simulink model "r2_b8a4x1kf"  (R2012b)
settings: Solver=VariableStepDiscrete  SolverMode=SingleTasking  StartTime=0.0  StopTime=1  RelTol=1e-3
undefined symbols (not defined in the file): fft_stages, n_bits_ants, n_bits_xengs
libraries: xbsIndex_r4 x22142, casper_library_misc x166, xbsReplacements_r4 x24, casper_library_delays x8, xps_library x5, casper_library_communications x4
(part 130 of 178)

== system r2_b8a4x1kf/sys3/xeng/baseline_tap3/dual_pol_cmac/cmac2 ==
  a+bi : Inport
  c+di : Inport  Port=2
  acc_in : Inport  Port=3
  sync : Inport  Port=4
  valid_in : Inport  Port=5
  Constant1 : xbsIndex_r4/Constant  const=0  gui_display_data_type=Fixed-point  arith_type=Unsigned  n_bits=bit_growth  bin_pt=0  preci_type=Single  exp_width=8  frac_width=24  explicit_period=on  period=1  equ=P=C  opselect=C  inp2=PCIN>>17  opr=+  inp1=P  carry=CIN  dbl_ovrd=off  block_type=constant
      settings: block_version=9.2.01
  Constant2 : xbsIndex_r4/Constant  const=0  gui_display_data_type=Fixed-point  arith_type=Unsigned  n_bits=1  bin_pt=0  preci_type=Single  exp_width=8  frac_width=24  explicit_period=off  period=1  equ=P=C  opselect=C  inp2=PCIN>>17  opr=+  inp1=P  carry=CIN  dbl_ovrd=off  block_type=constant
      settings: block_version=9.2.01
  Counter : xbsIndex_r4/Counter  cnt_type=Count Limited  cnt_to=acc_len - 1  operation=Up  start_count=0  cnt_by_val=1  arith_type=Unsigned  n_bits=bit_growth  bin_pt=0  load_pin=off  rst=on  en=off  explicit_period=off  period=1  dbl_ovrd=off  use_behavioral_HDL=off  implementation=Fabric  use_rpm=on  block_type=counter
      settings: xl_area=[0, 0, 0, 0, 0, 0, 0]  block_version=9.2.01
  Delay : xbsIndex_r4/Delay  rst=off  infoeditControl=Selection of Reset will increase slice count due to use of real FFs and instead of SRLs  en=off  latency=add_latency + mult_latency - 1  dbl_ovrd=off  reg_retiming=on  block_type=delay
      settings: xl_area=[0, 0, 0, 0, 0, 0, 0]  block_version=9.2.01
  Relational : xbsIndex_r4/Relational  mode=a=b  en=off  latency=1  dbl_ovrd=off  block_type=relational
      settings: xl_area=[0, 0, 0, 0, 0, 0, 0]  block_version=9.2.01
  Terminator : Terminator
  acc : Subsystem
  acc1 : Subsystem
  c_to_ri1 : Subsystem
  c_to_ri2 : Subsystem
  cmult* : Subsystem  AncestorBlock=casper_library_multipliers/cmult  mask(cmult){n_bits_a=8, bin_pt_a=7, n_bits_b=8, bin_pt_b=7, n_bits_ab=25, bin_pt_ab=14, quantization=Truncate, overflow=Wrap, in_latency=0, mult_latency=4, add_latency=3, conv_latency=0, conjugated=on, async=off, pipelined_enable=on, multiplier_implementation=embedded multiplier core}
      mask prompts: n_bits_a "Number of Bits 'a'"; bin_pt_a "Binary Point 'a'"; n_bits_b "Number of Bits 'b'"; bin_pt_b "Binary Point 'b'"; n_bits_ab "Number of Bits 'ab'"; bin_pt_ab "Binary Point 'ab'"; in_latency "Input latency"; mult_latency "Multiplier Latency"; add_latency "Adder Latency"; conv_latency "Convert latency"; conjugated "Conjugate"; async "asynchronous operation"; pipelined_enable "enable pipeline"; multiplier_implementation "Multiplier implementation"
      mask help:
      | Multiplies two complex numbers using 4 multipliers and 2 adders.
      | Conjugation is optional.
      mask init: same as r2_b8a4x1kf/sys0/xeng/auto_tap/dual_pol_cmac/cmac1/cmult*
      settings: AttributesFormatString=|
      | 8_7 * 8_7 ==> 25_14
      | Truncate, Wrap
      | Latency=0
      mask TypeOptions quantization: Truncate | Round  (unbiased: +/- Inf) | Round  (unbiased: Even Values)
      mask TypeOptions overflow: Wrap | Saturate | Flag as error
      mask TypeOptions multiplier_implementation: behavioral HDL | standard core | embedded multiplier core
  ri_to_c : Subsystem
  acc_out : Outport
  valid_out : Outport  Port=2
  wires:
  cmult*/1(ab) -> c_to_ri1/1(In1)
  valid_in/1 -> acc1/4(valid_in)
  acc1/2(valid_out) -> valid_out/1
  acc/2(valid_out) -> Terminator/1
  Constant2/1 -> acc/4(valid_in)
  Delay/1 -> Counter/1
  sync/1 -> Delay/1
  Constant1/1 -> Relational/2
  Counter/1 -> Relational/1
  Relational/1 -> acc1/1(rst), acc/1(rst)
  c_to_ri2/2(Out2) -> acc1/3(acc_in)
  ri_to_c/1(Out1) -> acc_out/1
  acc1/1(acc_out) -> ri_to_c/2(In2)
  acc_in/1 -> c_to_ri2/1(In1)
  c+di/1 -> cmult*/2(b)
  a+bi/1 -> cmult*/1(a)
  c_to_ri1/1(Out1) -> acc/2(din)  "auto_real"
  c_to_ri1/2(Out2) -> acc1/2(din)
  acc/1(acc_out) -> ri_to_c/1(In1)
  c_to_ri2/1(Out1) -> acc/3(acc_in)

== system r2_b8a4x1kf/sys3/xeng/baseline_tap3/dual_pol_cmac/cmac3 ==
  a+bi : Inport
  c+di : Inport  Port=2
  acc_in : Inport  Port=3
  sync : Inport  Port=4
  valid_in : Inport  Port=5
  Constant1 : xbsIndex_r4/Constant  const=0  gui_display_data_type=Fixed-point  arith_type=Unsigned  n_bits=bit_growth  bin_pt=0  preci_type=Single  exp_width=8  frac_width=24  explicit_period=on  period=1  equ=P=C  opselect=C  inp2=PCIN>>17  opr=+  inp1=P  carry=CIN  dbl_ovrd=off  block_type=constant
      settings: block_version=9.2.01
  Constant2 : xbsIndex_r4/Constant  const=0  gui_display_data_type=Fixed-point  arith_type=Unsigned  n_bits=1  bin_pt=0  preci_type=Single  exp_width=8  frac_width=24  explicit_period=off  period=1  equ=P=C  opselect=C  inp2=PCIN>>17  opr=+  inp1=P  carry=CIN  dbl_ovrd=off  block_type=constant
      settings: block_version=9.2.01
  Counter : xbsIndex_r4/Counter  cnt_type=Count Limited  cnt_to=acc_len - 1  operation=Up  start_count=0  cnt_by_val=1  arith_type=Unsigned  n_bits=bit_growth  bin_pt=0  load_pin=off  rst=on  en=off  explicit_period=off  period=1  dbl_ovrd=off  use_behavioral_HDL=off  implementation=Fabric  use_rpm=on  block_type=counter
      settings: xl_area=[0, 0, 0, 0, 0, 0, 0]  block_version=9.2.01
  Delay : xbsIndex_r4/Delay  rst=off  infoeditControl=Selection of Reset will increase slice count due to use of real FFs and instead of SRLs  en=off  latency=add_latency + mult_latency - 1  dbl_ovrd=off  reg_retiming=on  block_type=delay
      settings: xl_area=[0, 0, 0, 0, 0, 0, 0]  block_version=9.2.01
  Relational : xbsIndex_r4/Relational  mode=a=b  en=off  latency=1  dbl_ovrd=off  block_type=relational
      settings: xl_area=[0, 0, 0, 0, 0, 0, 0]  block_version=9.2.01
  Terminator : Terminator
  acc : Subsystem
  acc1 : Subsystem
  c_to_ri1 : Subsystem
  c_to_ri2 : Subsystem
  cmult* : Subsystem  AncestorBlock=casper_library_multipliers/cmult  mask(cmult){n_bits_a=8, bin_pt_a=7, n_bits_b=8, bin_pt_b=7, n_bits_ab=25, bin_pt_ab=14, quantization=Truncate, overflow=Wrap, in_latency=0, mult_latency=4, add_latency=3, conv_latency=0, conjugated=on, async=off, pipelined_enable=on, multiplier_implementation=embedded multiplier core}
      mask prompts: n_bits_a "Number of Bits 'a'"; bin_pt_a "Binary Point 'a'"; n_bits_b "Number of Bits 'b'"; bin_pt_b "Binary Point 'b'"; n_bits_ab "Number of Bits 'ab'"; bin_pt_ab "Binary Point 'ab'"; in_latency "Input latency"; mult_latency "Multiplier Latency"; add_latency "Adder Latency"; conv_latency "Convert latency"; conjugated "Conjugate"; async "asynchronous operation"; pipelined_enable "enable pipeline"; multiplier_implementation "Multiplier implementation"
      mask help:
      | Multiplies two complex numbers using 4 multipliers and 2 adders.
      | Conjugation is optional.
      mask init: same as r2_b8a4x1kf/sys0/xeng/auto_tap/dual_pol_cmac/cmac1/cmult*
      settings: AttributesFormatString=|
      | 8_7 * 8_7 ==> 25_14
      | Truncate, Wrap
      | Latency=0
      mask TypeOptions quantization: Truncate | Round  (unbiased: +/- Inf) | Round  (unbiased: Even Values)
      mask TypeOptions overflow: Wrap | Saturate | Flag as error
      mask TypeOptions multiplier_implementation: behavioral HDL | standard core | embedded multiplier core
  ri_to_c : Subsystem
  acc_out : Outport
  valid_out : Outport  Port=2
  wires:
  cmult*/1(ab) -> c_to_ri1/1(In1)
  valid_in/1 -> acc1/4(valid_in)
  acc1/2(valid_out) -> valid_out/1
  acc/2(valid_out) -> Terminator/1
  Constant2/1 -> acc/4(valid_in)
  Delay/1 -> Counter/1
  sync/1 -> Delay/1
  Constant1/1 -> Relational/2
  Counter/1 -> Relational/1
  Relational/1 -> acc1/1(rst), acc/1(rst)
  c_to_ri2/2(Out2) -> acc1/3(acc_in)
  ri_to_c/1(Out1) -> acc_out/1
  acc1/1(acc_out) -> ri_to_c/2(In2)
  acc_in/1 -> c_to_ri2/1(In1)
  c+di/1 -> cmult*/2(b)
  a+bi/1 -> cmult*/1(a)
  c_to_ri1/1(Out1) -> acc/2(din)  "auto_real"
  c_to_ri1/2(Out2) -> acc1/2(din)
  acc/1(acc_out) -> ri_to_c/1(In1)
  c_to_ri2/1(Out1) -> acc/3(acc_in)

== system r2_b8a4x1kf/sys3/xeng/baseline_tap3/dual_pol_cmac/cmac4 ==
  a+bi : Inport
  c+di : Inport  Port=2
  acc_in : Inport  Port=3
  sync : Inport  Port=4
  valid_in : Inport  Port=5
  Constant1 : xbsIndex_r4/Constant  const=0  gui_display_data_type=Fixed-point  arith_type=Unsigned  n_bits=bit_growth  bin_pt=0  preci_type=Single  exp_width=8  frac_width=24  explicit_period=on  period=1  equ=P=C  opselect=C  inp2=PCIN>>17  opr=+  inp1=P  carry=CIN  dbl_ovrd=off  block_type=constant
      settings: block_version=9.2.01
  Constant2 : xbsIndex_r4/Constant  const=0  gui_display_data_type=Fixed-point  arith_type=Unsigned  n_bits=1  bin_pt=0  preci_type=Single  exp_width=8  frac_width=24  explicit_period=off  period=1  equ=P=C  opselect=C  inp2=PCIN>>17  opr=+  inp1=P  carry=CIN  dbl_ovrd=off  block_type=constant
      settings: block_version=9.2.01
  Counter : xbsIndex_r4/Counter  cnt_type=Count Limited  cnt_to=acc_len - 1  operation=Up  start_count=0  cnt_by_val=1  arith_type=Unsigned  n_bits=bit_growth  bin_pt=0  load_pin=off  rst=on  en=off  explicit_period=off  period=1  dbl_ovrd=off  use_behavioral_HDL=off  implementation=Fabric  use_rpm=on  block_type=counter
      settings: xl_area=[0, 0, 0, 0, 0, 0, 0]  block_version=9.2.01
  Delay : xbsIndex_r4/Delay  rst=off  infoeditControl=Selection of Reset will increase slice count due to use of real FFs and instead of SRLs  en=off  latency=add_latency + mult_latency - 1  dbl_ovrd=off  reg_retiming=on  block_type=delay
      settings: xl_area=[0, 0, 0, 0, 0, 0, 0]  block_version=9.2.01
  Relational : xbsIndex_r4/Relational  mode=a=b  en=off  latency=1  dbl_ovrd=off  block_type=relational
      settings: xl_area=[0, 0, 0, 0, 0, 0, 0]  block_version=9.2.01
  Terminator : Terminator
  acc : Subsystem
  acc1 : Subsystem
  c_to_ri1 : Subsystem
  c_to_ri2 : Subsystem
  cmult* : Subsystem  AncestorBlock=casper_library_multipliers/cmult  mask(cmult){n_bits_a=8, bin_pt_a=7, n_bits_b=8, bin_pt_b=7, n_bits_ab=25, bin_pt_ab=14, quantization=Truncate, overflow=Wrap, in_latency=0, mult_latency=4, add_latency=3, conv_latency=0, conjugated=on, async=off, pipelined_enable=on, multiplier_implementation=embedded multiplier core}
      mask prompts: n_bits_a "Number of Bits 'a'"; bin_pt_a "Binary Point 'a'"; n_bits_b "Number of Bits 'b'"; bin_pt_b "Binary Point 'b'"; n_bits_ab "Number of Bits 'ab'"; bin_pt_ab "Binary Point 'ab'"; in_latency "Input latency"; mult_latency "Multiplier Latency"; add_latency "Adder Latency"; conv_latency "Convert latency"; conjugated "Conjugate"; async "asynchronous operation"; pipelined_enable "enable pipeline"; multiplier_implementation "Multiplier implementation"
      mask help:
      | Multiplies two complex numbers using 4 multipliers and 2 adders.
      | Conjugation is optional.
      mask init: same as r2_b8a4x1kf/sys0/xeng/auto_tap/dual_pol_cmac/cmac1/cmult*
      settings: AttributesFormatString=|
      | 8_7 * 8_7 ==> 25_14
      | Truncate, Wrap
      | Latency=0
      mask TypeOptions quantization: Truncate | Round  (unbiased: +/- Inf) | Round  (unbiased: Even Values)
      mask TypeOptions overflow: Wrap | Saturate | Flag as error
      mask TypeOptions multiplier_implementation: behavioral HDL | standard core | embedded multiplier core
  ri_to_c : Subsystem
  acc_out : Outport
  valid_out : Outport  Port=2
  wires:
  cmult*/1(ab) -> c_to_ri1/1(In1)
  valid_in/1 -> acc1/4(valid_in)
  acc1/2(valid_out) -> valid_out/1
  acc/2(valid_out) -> Terminator/1
  Constant2/1 -> acc/4(valid_in)
  Delay/1 -> Counter/1
  sync/1 -> Delay/1
  Constant1/1 -> Relational/2
  Counter/1 -> Relational/1
  Relational/1 -> acc1/1(rst), acc/1(rst)
  c_to_ri2/2(Out2) -> acc1/3(acc_in)
  ri_to_c/1(Out1) -> acc_out/1
  acc1/1(acc_out) -> ri_to_c/2(In2)
  acc_in/1 -> c_to_ri2/1(In1)
  c+di/1 -> cmult*/2(b)
  a+bi/1 -> cmult*/1(a)
  c_to_ri1/1(Out1) -> acc/2(din)  "auto_real"
  c_to_ri1/2(Out2) -> acc1/2(din)
  acc/1(acc_out) -> ri_to_c/1(In1)
  c_to_ri2/1(Out1) -> acc/3(acc_in)

== system r2_b8a4x1kf/sys3/xeng/baseline_tap4/dual_pol_cmac/cmac1 ==
  a+bi : Inport
  c+di : Inport  Port=2
  acc_in : Inport  Port=3
  sync : Inport  Port=4
  valid_in : Inport  Port=5
  Constant1 : xbsIndex_r4/Constant  const=0  gui_display_data_type=Fixed-point  arith_type=Unsigned  n_bits=bit_growth  bin_pt=0  preci_type=Single  exp_width=8  frac_width=24  explicit_period=on  period=1  equ=P=C  opselect=C  inp2=PCIN>>17  opr=+  inp1=P  carry=CIN  dbl_ovrd=off  block_type=constant
      settings: block_version=9.2.01
  Constant2 : xbsIndex_r4/Constant  const=0  gui_display_data_type=Fixed-point  arith_type=Unsigned  n_bits=1  bin_pt=0  preci_type=Single  exp_width=8  frac_width=24  explicit_period=off  period=1  equ=P=C  opselect=C  inp2=PCIN>>17  opr=+  inp1=P  carry=CIN  dbl_ovrd=off  block_type=constant
      settings: block_version=9.2.01
  Counter : xbsIndex_r4/Counter  cnt_type=Count Limited  cnt_to=acc_len - 1  operation=Up  start_count=0  cnt_by_val=1  arith_type=Unsigned  n_bits=bit_growth  bin_pt=0  load_pin=off  rst=on  en=off  explicit_period=off  period=1  dbl_ovrd=off  use_behavioral_HDL=off  implementation=Fabric  use_rpm=on  block_type=counter
      settings: xl_area=[0, 0, 0, 0, 0, 0, 0]  block_version=9.2.01
  Delay : xbsIndex_r4/Delay  rst=off  infoeditControl=Selection of Reset will increase slice count due to use of real FFs and instead of SRLs  en=off  latency=add_latency + mult_latency - 1  dbl_ovrd=off  reg_retiming=on  block_type=delay
      settings: xl_area=[0, 0, 0, 0, 0, 0, 0]  block_version=9.2.01
  Relational : xbsIndex_r4/Relational  mode=a=b  en=off  latency=1  dbl_ovrd=off  block_type=relational
      settings: xl_area=[0, 0, 0, 0, 0, 0, 0]  block_version=9.2.01
  Terminator : Terminator
  acc : Subsystem
  acc1 : Subsystem
  c_to_ri1 : Subsystem
  c_to_ri2 : Subsystem
  cmult* : Subsystem  AncestorBlock=casper_library_multipliers/cmult  mask(cmult){n_bits_a=8, bin_pt_a=7, n_bits_b=8, bin_pt_b=7, n_bits_ab=25, bin_pt_ab=14, quantization=Truncate, overflow=Wrap, in_latency=0, mult_latency=4, add_latency=3, conv_latency=0, conjugated=on, async=off, pipelined_enable=on, multiplier_implementation=embedded multiplier core}
      mask prompts: n_bits_a "Number of Bits 'a'"; bin_pt_a "Binary Point 'a'"; n_bits_b "Number of Bits 'b'"; bin_pt_b "Binary Point 'b'"; n_bits_ab "Number of Bits 'ab'"; bin_pt_ab "Binary Point 'ab'"; in_latency "Input latency"; mult_latency "Multiplier Latency"; add_latency "Adder Latency"; conv_latency "Convert latency"; conjugated "Conjugate"; async "asynchronous operation"; pipelined_enable "enable pipeline"; multiplier_implementation "Multiplier implementation"
      mask help:
      | Multiplies two complex numbers using 4 multipliers and 2 adders.
      | Conjugation is optional.
      mask init: same as r2_b8a4x1kf/sys0/xeng/auto_tap/dual_pol_cmac/cmac1/cmult*
      settings: AttributesFormatString=|
      | 8_7 * 8_7 ==> 25_14
      | Truncate, Wrap
      | Latency=0
      mask TypeOptions quantization: Truncate | Round  (unbiased: +/- Inf) | Round  (unbiased: Even Values)
      mask TypeOptions overflow: Wrap | Saturate | Flag as error
      mask TypeOptions multiplier_implementation: behavioral HDL | standard core | embedded multiplier core
  ri_to_c : Subsystem
  acc_out : Outport
  valid_out : Outport  Port=2
  wires:
  cmult*/1(ab) -> c_to_ri1/1(In1)
  valid_in/1 -> acc1/4(valid_in)
  acc1/2(valid_out) -> valid_out/1
  acc/2(valid_out) -> Terminator/1
  Constant2/1 -> acc/4(valid_in)
  Delay/1 -> Counter/1
  sync/1 -> Delay/1
  Constant1/1 -> Relational/2
  Counter/1 -> Relational/1
  Relational/1 -> acc1/1(rst), acc/1(rst)
  c_to_ri2/2(Out2) -> acc1/3(acc_in)
  ri_to_c/1(Out1) -> acc_out/1
  acc1/1(acc_out) -> ri_to_c/2(In2)
  acc_in/1 -> c_to_ri2/1(In1)
  c+di/1 -> cmult*/2(b)
  a+bi/1 -> cmult*/1(a)
  c_to_ri1/1(Out1) -> acc/2(din)  "auto_real"
  c_to_ri1/2(Out2) -> acc1/2(din)
  acc/1(acc_out) -> ri_to_c/1(In1)
  c_to_ri2/1(Out1) -> acc/3(acc_in)

== system r2_b8a4x1kf/sys3/xeng/baseline_tap4/dual_pol_cmac/cmac2 ==
  a+bi : Inport
  c+di : Inport  Port=2
  acc_in : Inport  Port=3
  sync : Inport  Port=4
  valid_in : Inport  Port=5
  Constant1 : xbsIndex_r4/Constant  const=0  gui_display_data_type=Fixed-point  arith_type=Unsigned  n_bits=bit_growth  bin_pt=0  preci_type=Single  exp_width=8  frac_width=24  explicit_period=on  period=1  equ=P=C  opselect=C  inp2=PCIN>>17  opr=+  inp1=P  carry=CIN  dbl_ovrd=off  block_type=constant
      settings: block_version=9.2.01
  Constant2 : xbsIndex_r4/Constant  const=0  gui_display_data_type=Fixed-point  arith_type=Unsigned  n_bits=1  bin_pt=0  preci_type=Single  exp_width=8  frac_width=24  explicit_period=off  period=1  equ=P=C  opselect=C  inp2=PCIN>>17  opr=+  inp1=P  carry=CIN  dbl_ovrd=off  block_type=constant
      settings: block_version=9.2.01
  Counter : xbsIndex_r4/Counter  cnt_type=Count Limited  cnt_to=acc_len - 1  operation=Up  start_count=0  cnt_by_val=1  arith_type=Unsigned  n_bits=bit_growth  bin_pt=0  load_pin=off  rst=on  en=off  explicit_period=off  period=1  dbl_ovrd=off  use_behavioral_HDL=off  implementation=Fabric  use_rpm=on  block_type=counter
      settings: xl_area=[0, 0, 0, 0, 0, 0, 0]  block_version=9.2.01
  Delay : xbsIndex_r4/Delay  rst=off  infoeditControl=Selection of Reset will increase slice count due to use of real FFs and instead of SRLs  en=off  latency=add_latency + mult_latency - 1  dbl_ovrd=off  reg_retiming=on  block_type=delay
      settings: xl_area=[0, 0, 0, 0, 0, 0, 0]  block_version=9.2.01
  Relational : xbsIndex_r4/Relational  mode=a=b  en=off  latency=1  dbl_ovrd=off  block_type=relational
      settings: xl_area=[0, 0, 0, 0, 0, 0, 0]  block_version=9.2.01
  Terminator : Terminator
  acc : Subsystem
  acc1 : Subsystem
  c_to_ri1 : Subsystem
  c_to_ri2 : Subsystem
  cmult* : Subsystem  AncestorBlock=casper_library_multipliers/cmult  mask(cmult){n_bits_a=8, bin_pt_a=7, n_bits_b=8, bin_pt_b=7, n_bits_ab=25, bin_pt_ab=14, quantization=Truncate, overflow=Wrap, in_latency=0, mult_latency=4, add_latency=3, conv_latency=0, conjugated=on, async=off, pipelined_enable=on, multiplier_implementation=embedded multiplier core}
      mask prompts: n_bits_a "Number of Bits 'a'"; bin_pt_a "Binary Point 'a'"; n_bits_b "Number of Bits 'b'"; bin_pt_b "Binary Point 'b'"; n_bits_ab "Number of Bits 'ab'"; bin_pt_ab "Binary Point 'ab'"; in_latency "Input latency"; mult_latency "Multiplier Latency"; add_latency "Adder Latency"; conv_latency "Convert latency"; conjugated "Conjugate"; async "asynchronous operation"; pipelined_enable "enable pipeline"; multiplier_implementation "Multiplier implementation"
      mask help:
      | Multiplies two complex numbers using 4 multipliers and 2 adders.
      | Conjugation is optional.
      mask init: same as r2_b8a4x1kf/sys0/xeng/auto_tap/dual_pol_cmac/cmac1/cmult*
      settings: AttributesFormatString=|
      | 8_7 * 8_7 ==> 25_14
      | Truncate, Wrap
      | Latency=0
      mask TypeOptions quantization: Truncate | Round  (unbiased: +/- Inf) | Round  (unbiased: Even Values)
      mask TypeOptions overflow: Wrap | Saturate | Flag as error
      mask TypeOptions multiplier_implementation: behavioral HDL | standard core | embedded multiplier core
  ri_to_c : Subsystem
  acc_out : Outport
  valid_out : Outport  Port=2
  wires:
  cmult*/1(ab) -> c_to_ri1/1(In1)
  valid_in/1 -> acc1/4(valid_in)
  acc1/2(valid_out) -> valid_out/1
  acc/2(valid_out) -> Terminator/1
  Constant2/1 -> acc/4(valid_in)
  Delay/1 -> Counter/1
  sync/1 -> Delay/1
  Constant1/1 -> Relational/2
  Counter/1 -> Relational/1
  Relational/1 -> acc1/1(rst), acc/1(rst)
  c_to_ri2/2(Out2) -> acc1/3(acc_in)
  ri_to_c/1(Out1) -> acc_out/1
  acc1/1(acc_out) -> ri_to_c/2(In2)
  acc_in/1 -> c_to_ri2/1(In1)
  c+di/1 -> cmult*/2(b)
  a+bi/1 -> cmult*/1(a)
  c_to_ri1/1(Out1) -> acc/2(din)  "auto_real"
  c_to_ri1/2(Out2) -> acc1/2(din)
  acc/1(acc_out) -> ri_to_c/1(In1)
  c_to_ri2/1(Out1) -> acc/3(acc_in)

== system r2_b8a4x1kf/sys3/xeng/baseline_tap4/dual_pol_cmac/cmac3 ==
  a+bi : Inport
  c+di : Inport  Port=2
  acc_in : Inport  Port=3
  sync : Inport  Port=4
  valid_in : Inport  Port=5
  Constant1 : xbsIndex_r4/Constant  const=0  gui_display_data_type=Fixed-point  arith_type=Unsigned  n_bits=bit_growth  bin_pt=0  preci_type=Single  exp_width=8  frac_width=24  explicit_period=on  period=1  equ=P=C  opselect=C  inp2=PCIN>>17  opr=+  inp1=P  carry=CIN  dbl_ovrd=off  block_type=constant
      settings: block_version=9.2.01
  Constant2 : xbsIndex_r4/Constant  const=0  gui_display_data_type=Fixed-point  arith_type=Unsigned  n_bits=1  bin_pt=0  preci_type=Single  exp_width=8  frac_width=24  explicit_period=off  period=1  equ=P=C  opselect=C  inp2=PCIN>>17  opr=+  inp1=P  carry=CIN  dbl_ovrd=off  block_type=constant
      settings: block_version=9.2.01
  Counter : xbsIndex_r4/Counter  cnt_type=Count Limited  cnt_to=acc_len - 1  operation=Up  start_count=0  cnt_by_val=1  arith_type=Unsigned  n_bits=bit_growth  bin_pt=0  load_pin=off  rst=on  en=off  explicit_period=off  period=1  dbl_ovrd=off  use_behavioral_HDL=off  implementation=Fabric  use_rpm=on  block_type=counter
      settings: xl_area=[0, 0, 0, 0, 0, 0, 0]  block_version=9.2.01
  Delay : xbsIndex_r4/Delay  rst=off  infoeditControl=Selection of Reset will increase slice count due to use of real FFs and instead of SRLs  en=off  latency=add_latency + mult_latency - 1  dbl_ovrd=off  reg_retiming=on  block_type=delay
      settings: xl_area=[0, 0, 0, 0, 0, 0, 0]  block_version=9.2.01
  Relational : xbsIndex_r4/Relational  mode=a=b  en=off  latency=1  dbl_ovrd=off  block_type=relational
      settings: xl_area=[0, 0, 0, 0, 0, 0, 0]  block_version=9.2.01
  Terminator : Terminator
  acc : Subsystem
  acc1 : Subsystem
  c_to_ri1 : Subsystem
  c_to_ri2 : Subsystem
  cmult* : Subsystem  AncestorBlock=casper_library_multipliers/cmult  mask(cmult){n_bits_a=8, bin_pt_a=7, n_bits_b=8, bin_pt_b=7, n_bits_ab=25, bin_pt_ab=14, quantization=Truncate, overflow=Wrap, in_latency=0, mult_latency=4, add_latency=3, conv_latency=0, conjugated=on, async=off, pipelined_enable=on, multiplier_implementation=embedded multiplier core}
      mask prompts: n_bits_a "Number of Bits 'a'"; bin_pt_a "Binary Point 'a'"; n_bits_b "Number of Bits 'b'"; bin_pt_b "Binary Point 'b'"; n_bits_ab "Number of Bits 'ab'"; bin_pt_ab "Binary Point 'ab'"; in_latency "Input latency"; mult_latency "Multiplier Latency"; add_latency "Adder Latency"; conv_latency "Convert latency"; conjugated "Conjugate"; async "asynchronous operation"; pipelined_enable "enable pipeline"; multiplier_implementation "Multiplier implementation"
      mask help:
      | Multiplies two complex numbers using 4 multipliers and 2 adders.
      | Conjugation is optional.
      mask init: same as r2_b8a4x1kf/sys0/xeng/auto_tap/dual_pol_cmac/cmac1/cmult*
      settings: AttributesFormatString=|
      | 8_7 * 8_7 ==> 25_14
      | Truncate, Wrap
      | Latency=0
      mask TypeOptions quantization: Truncate | Round  (unbiased: +/- Inf) | Round  (unbiased: Even Values)
      mask TypeOptions overflow: Wrap | Saturate | Flag as error
      mask TypeOptions multiplier_implementation: behavioral HDL | standard core | embedded multiplier core
  ri_to_c : Subsystem
  acc_out : Outport
  valid_out : Outport  Port=2
  wires:
  cmult*/1(ab) -> c_to_ri1/1(In1)
  valid_in/1 -> acc1/4(valid_in)
  acc1/2(valid_out) -> valid_out/1
  acc/2(valid_out) -> Terminator/1
  Constant2/1 -> acc/4(valid_in)
  Delay/1 -> Counter/1
  sync/1 -> Delay/1
  Constant1/1 -> Relational/2
  Counter/1 -> Relational/1
  Relational/1 -> acc1/1(rst), acc/1(rst)
  c_to_ri2/2(Out2) -> acc1/3(acc_in)
  ri_to_c/1(Out1) -> acc_out/1
  acc1/1(acc_out) -> ri_to_c/2(In2)
  acc_in/1 -> c_to_ri2/1(In1)
  c+di/1 -> cmult*/2(b)
  a+bi/1 -> cmult*/1(a)
  c_to_ri1/1(Out1) -> acc/2(din)  "auto_real"
  c_to_ri1/2(Out2) -> acc1/2(din)
  acc/1(acc_out) -> ri_to_c/1(In1)
  c_to_ri2/1(Out1) -> acc/3(acc_in)

== system r2_b8a4x1kf/sys3/xeng/baseline_tap4/dual_pol_cmac/cmac4 ==
  a+bi : Inport
  c+di : Inport  Port=2
  acc_in : Inport  Port=3
  sync : Inport  Port=4
  valid_in : Inport  Port=5
  Constant1 : xbsIndex_r4/Constant  const=0  gui_display_data_type=Fixed-point  arith_type=Unsigned  n_bits=bit_growth  bin_pt=0  preci_type=Single  exp_width=8  frac_width=24  explicit_period=on  period=1  equ=P=C  opselect=C  inp2=PCIN>>17  opr=+  inp1=P  carry=CIN  dbl_ovrd=off  block_type=constant
      settings: block_version=9.2.01
  Constant2 : xbsIndex_r4/Constant  const=0  gui_display_data_type=Fixed-point  arith_type=Unsigned  n_bits=1  bin_pt=0  preci_type=Single  exp_width=8  frac_width=24  explicit_period=off  period=1  equ=P=C  opselect=C  inp2=PCIN>>17  opr=+  inp1=P  carry=CIN  dbl_ovrd=off  block_type=constant
      settings: block_version=9.2.01
  Counter : xbsIndex_r4/Counter  cnt_type=Count Limited  cnt_to=acc_len - 1  operation=Up  start_count=0  cnt_by_val=1  arith_type=Unsigned  n_bits=bit_growth  bin_pt=0  load_pin=off  rst=on  en=off  explicit_period=off  period=1  dbl_ovrd=off  use_behavioral_HDL=off  implementation=Fabric  use_rpm=on  block_type=counter
      settings: xl_area=[0, 0, 0, 0, 0, 0, 0]  block_version=9.2.01
  Delay : xbsIndex_r4/Delay  rst=off  infoeditControl=Selection of Reset will increase slice count due to use of real FFs and instead of SRLs  en=off  latency=add_latency + mult_latency - 1  dbl_ovrd=off  reg_retiming=on  block_type=delay
      settings: xl_area=[0, 0, 0, 0, 0, 0, 0]  block_version=9.2.01
  Relational : xbsIndex_r4/Relational  mode=a=b  en=off  latency=1  dbl_ovrd=off  block_type=relational
      settings: xl_area=[0, 0, 0, 0, 0, 0, 0]  block_version=9.2.01
  Terminator : Terminator
  acc : Subsystem
  acc1 : Subsystem
  c_to_ri1 : Subsystem
  c_to_ri2 : Subsystem
  cmult* : Subsystem  AncestorBlock=casper_library_multipliers/cmult  mask(cmult){n_bits_a=8, bin_pt_a=7, n_bits_b=8, bin_pt_b=7, n_bits_ab=25, bin_pt_ab=14, quantization=Truncate, overflow=Wrap, in_latency=0, mult_latency=4, add_latency=3, conv_latency=0, conjugated=on, async=off, pipelined_enable=on, multiplier_implementation=embedded multiplier core}
      mask prompts: n_bits_a "Number of Bits 'a'"; bin_pt_a "Binary Point 'a'"; n_bits_b "Number of Bits 'b'"; bin_pt_b "Binary Point 'b'"; n_bits_ab "Number of Bits 'ab'"; bin_pt_ab "Binary Point 'ab'"; in_latency "Input latency"; mult_latency "Multiplier Latency"; add_latency "Adder Latency"; conv_latency "Convert latency"; conjugated "Conjugate"; async "asynchronous operation"; pipelined_enable "enable pipeline"; multiplier_implementation "Multiplier implementation"
      mask help:
      | Multiplies two complex numbers using 4 multipliers and 2 adders.
      | Conjugation is optional.
      mask init: same as r2_b8a4x1kf/sys0/xeng/auto_tap/dual_pol_cmac/cmac1/cmult*
      settings: AttributesFormatString=|
      | 8_7 * 8_7 ==> 25_14
      | Truncate, Wrap
      | Latency=0
      mask TypeOptions quantization: Truncate | Round  (unbiased: +/- Inf) | Round  (unbiased: Even Values)
      mask TypeOptions overflow: Wrap | Saturate | Flag as error
      mask TypeOptions multiplier_implementation: behavioral HDL | standard core | embedded multiplier core
  ri_to_c : Subsystem
  acc_out : Outport
  valid_out : Outport  Port=2
  wires:
  cmult*/1(ab) -> c_to_ri1/1(In1)
  valid_in/1 -> acc1/4(valid_in)
  acc1/2(valid_out) -> valid_out/1
  acc/2(valid_out) -> Terminator/1
  Constant2/1 -> acc/4(valid_in)
  Delay/1 -> Counter/1
  sync/1 -> Delay/1
  Constant1/1 -> Relational/2
  Counter/1 -> Relational/1
  Relational/1 -> acc1/1(rst), acc/1(rst)
  c_to_ri2/2(Out2) -> acc1/3(acc_in)
  ri_to_c/1(Out1) -> acc_out/1
  acc1/1(acc_out) -> ri_to_c/2(In2)
  acc_in/1 -> c_to_ri2/1(In1)
  c+di/1 -> cmult*/2(b)
  a+bi/1 -> cmult*/1(a)
  c_to_ri1/1(Out1) -> acc/2(din)  "auto_real"
  c_to_ri1/2(Out2) -> acc1/2(din)
  acc/1(acc_out) -> ri_to_c/1(In1)
  c_to_ri2/1(Out1) -> acc/3(acc_in)

== system r2_b8a4x1kf/sys3/xeng/xeng_descramble/write_ctrl/negedge_delay ==
  in : Inport
  Constant5 : xbsIndex_r4/Constant  const=pulse_len-2  gui_display_data_type=Fixed-point  arith_type=Unsigned  n_bits=bits  bin_pt=0  preci_type=Single  exp_width=8  frac_width=24  explicit_period=off  period=1  equ=P=C  opselect=C  inp2=PCIN>>17  opr=+  inp1=P  carry=CIN  dbl_ovrd=off  block_type=constant
      settings: block_version=9.1.01
  Counter3 : xbsIndex_r4/Counter  cnt_type=Free Running  cnt_to=1023  operation=Up  start_count=0  cnt_by_val=1  arith_type=Unsigned  n_bits=bits  bin_pt=0  load_pin=off  rst=on  en=on  explicit_period=on  period=1  dbl_ovrd=off  use_behavioral_HDL=off  implementation=Fabric  use_rpm=on  block_type=counter
      settings: xl_area=[0, 0, 0, 0, 0, 0, 0]  block_version=9.1.01
  Delay : xbsIndex_r4/Delay  rst=off  infoeditControl=Selection of Reset will increase slice count due to use of real FFs and instead of SRLs  en=off  latency=1  dbl_ovrd=off  reg_retiming=on  block_type=delay
  Logical : xbsIndex_r4/Logical  logical_function=OR  inputs=3  en=off  latency=0  precision=Full  arith_type=Unsigned  n_bits=16  bin_pt=0  align_bp=on  dbl_ovrd=off  block_type=logical
  Relational5 : xbsIndex_r4/Relational  mode=a<=b  en=off  latency=0  dbl_ovrd=off  block_type=relational
      settings: xl_area=[0, 0, 0, 0, 0, 0, 0]  block_version=9.1.01
  negedge : Subsystem  AncestorBlock=casper_library_misc/edge_detect  mask(edge_detect){edge=Falling, polarity=Active High, x_in=[0 0.08 0.08 0.16 0.16 0.24 0.24 0.32 0.32 0.4], y_in=[1  1 -1 -1 -1 -1 -1 -1 -1 -1], x_out=[0.6 0.68 0.68 0.76 0.76 0.84 0.84 0.92 0.92 1], y_out=[-1 -1  1  1 -1 -1 -1 -1 -1 -1]}
      mask prompts: edge "Edge Type"; polarity "Output Polarity"; x_in "Input X Positions"; y_in "Input Y Positions"; x_out "Output X Positions"; y_out "Output Y Positions"
      mask help: Output is active for one-cycle after each edge of the specified type (i.e. rising, falling or both).
      mask init: same as r2_b8a4x1kf/edge_detect
      settings: AttributesFormatString=|
      | falling edges
      | active high
      mask Help: Output is active for one-cycle after each edge of the specified type (i.e. rising, falling, or both).  Latency is zero.
      mask TypeOptions edge: Rising | Falling | Both
      mask TypeOptions polarity: Active High | Active Low
      mask Display:
      | plot(x_in_num,0.5+y_in_num*0.2);
      | plot(x_out_num,0.5+y_out_num*0.2);
  out : Outport
  wires:
  Delay/1 -> Logical/2
  Logical/1 -> out/1
  Counter3/1 -> Relational5/1
  Constant5/1 -> Relational5/2
  Relational5/1 -> Logical/3, Counter3/2
  in/1 -> negedge/1(in), Logical/1, Delay/1
  negedge/1(out) -> Counter3/1

== system r2_b8a4x1kf/bfsnap_out/ss/bram/mem/sim_munge_in/join ==
  in1 : Inport
  in2 : Inport  Port=2
  concatenate : xbsIndex_r4/Concat  num_inputs=2  dbl_ovrd=off  block_type=concat
  reinterpret1 : xbsIndex_r4/Reinterpret  force_arith_type=on  arith_type=Unsigned  force_bin_pt=on  bin_pt=0  block_type=reinterpret
      settings: infoedit="Changes signal type without altering the binary representation.   You can changed the signal between signed and unsigned, and relocate the binary point.<br><br>Hardware notes: In hardware this block costs nothing.<br><br>Example:  Suppose the input is 6 bits wide, signed, with 2 fractional bits, and the output is forced to unsigned with 0 fractional bits.  Then an input of -2.0 (1110.00 in binary 2's complement) becomes an output of 56 (111000 in binary)."
  reinterpret2 : xbsIndex_r4/Reinterpret  force_arith_type=on  arith_type=Unsigned  force_bin_pt=on  bin_pt=0  block_type=reinterpret
      settings: infoedit="Changes signal type without altering the binary representation.   You can changed the signal between signed and unsigned, and relocate the binary point.<br><br>Hardware notes: In hardware this block costs nothing.<br><br>Example:  Suppose the input is 6 bits wide, signed, with 2 fractional bits, and the output is forced to unsigned with 0 fractional bits.  Then an input of -2.0 (1110.00 in binary 2's complement) becomes an output of 56 (111000 in binary)."
  bus_out : Outport
  wires:
  concatenate/1 -> bus_out/1
  in1/1 -> reinterpret1/1
  reinterpret1/1 -> concatenate/1
  in2/1 -> reinterpret2/1
  reinterpret2/1 -> concatenate/2

== system r2_b8a4x1kf/bfsnap_out/ss/bram/mem/sim_munge_in/split ==
  bus_in : Inport
  reinterpret1 : xbsIndex_r4/Reinterpret  force_arith_type=on  arith_type=Unsigned  force_bin_pt=on  bin_pt=0  block_type=reinterpret
  reinterpret2 : xbsIndex_r4/Reinterpret  force_arith_type=on  arith_type=Unsigned  force_bin_pt=on  bin_pt=0  block_type=reinterpret
  slice1 : xbsIndex_r4/Slice  nbits=32  boolean_output=off  mode=Upper Bit Location + Width  bit1=-32  base1=MSB of Input  bit0=0  base0=LSB of Input  dbl_ovrd=off  block_type=slice
  slice2 : xbsIndex_r4/Slice  nbits=32  boolean_output=off  mode=Upper Bit Location + Width  bit1=0  base1=MSB of Input  bit0=0  base0=LSB of Input  dbl_ovrd=off  block_type=slice
  msb_out2 : Outport
  lsb_out1 : Outport  Port=2
  wires:
  reinterpret1/1 -> lsb_out1/1
  slice1/1 -> reinterpret1/1
  reinterpret2/1 -> msb_out2/1
  slice2/1 -> reinterpret2/1
  bus_in/1 -> slice1/1, slice2/1

== system r2_b8a4x1kf/bfsnap_out/ss/bram/mem/sim_munge_out/join ==
  in1 : Inport
  in2 : Inport  Port=2
  concatenate : xbsIndex_r4/Concat  num_inputs=2  dbl_ovrd=off  block_type=concat
  reinterpret1 : xbsIndex_r4/Reinterpret  force_arith_type=on  arith_type=Unsigned  force_bin_pt=on  bin_pt=0  block_type=reinterpret
      settings: infoedit="Changes signal type without altering the binary representation.   You can changed the signal between signed and unsigned, and relocate the binary point.<br><br>Hardware notes: In hardware this block costs nothing.<br><br>Example:  Suppose the input is 6 bits wide, signed, with 2 fractional bits, and the output is forced to unsigned with 0 fractional bits.  Then an input of -2.0 (1110.00 in binary 2's complement) becomes an output of 56 (111000 in binary)."
  reinterpret2 : xbsIndex_r4/Reinterpret  force_arith_type=on  arith_type=Unsigned  force_bin_pt=on  bin_pt=0  block_type=reinterpret
      settings: infoedit="Changes signal type without altering the binary representation.   You can changed the signal between signed and unsigned, and relocate the binary point.<br><br>Hardware notes: In hardware this block costs nothing.<br><br>Example:  Suppose the input is 6 bits wide, signed, with 2 fractional bits, and the output is forced to unsigned with 0 fractional bits.  Then an input of -2.0 (1110.00 in binary 2's complement) becomes an output of 56 (111000 in binary)."
  bus_out : Outport
  wires:
  concatenate/1 -> bus_out/1
  in1/1 -> reinterpret1/1
  reinterpret1/1 -> concatenate/1
  in2/1 -> reinterpret2/1
  reinterpret2/1 -> concatenate/2

== system r2_b8a4x1kf/bfsnap_out/ss/bram/mem/sim_munge_out/split ==
  bus_in : Inport
  reinterpret1 : xbsIndex_r4/Reinterpret  force_arith_type=on  arith_type=Unsigned  force_bin_pt=on  bin_pt=0  block_type=reinterpret
  reinterpret2 : xbsIndex_r4/Reinterpret  force_arith_type=on  arith_type=Unsigned  force_bin_pt=on  bin_pt=0  block_type=reinterpret
  slice1 : xbsIndex_r4/Slice  nbits=32  boolean_output=off  mode=Upper Bit Location + Width  bit1=-32  base1=MSB of Input  bit0=0  base0=LSB of Input  dbl_ovrd=off  block_type=slice
  slice2 : xbsIndex_r4/Slice  nbits=32  boolean_output=off  mode=Upper Bit Location + Width  bit1=0  base1=MSB of Input  bit0=0  base0=LSB of Input  dbl_ovrd=off  block_type=slice
  msb_out2 : Outport
  lsb_out1 : Outport  Port=2
  wires:
  reinterpret1/1 -> lsb_out1/1
  slice1/1 -> reinterpret1/1
  reinterpret2/1 -> msb_out2/1
  slice2/1 -> reinterpret2/1
  bus_in/1 -> slice1/1, slice2/1

== system r2_b8a4x1kf/sys0/bf/fbf/apply_beam_weights/munge_in/join ==
  in1 : Inport
  in2 : Inport  Port=2
  concatenate : xbsIndex_r4/Concat  num_inputs=2  dbl_ovrd=off  block_type=concat
  reinterpret1 : xbsIndex_r4/Reinterpret  force_arith_type=on  arith_type=Unsigned  force_bin_pt=on  bin_pt=0  block_type=reinterpret
      settings: infoedit="Changes signal type without altering the binary representation.   You can changed the signal between signed and unsigned, and relocate the binary point.<br><br>Hardware notes: In hardware this block costs nothing.<br><br>Example:  Suppose the input is 6 bits wide, signed, with 2 fractional bits, and the output is forced to unsigned with 0 fractional bits.  Then an input of -2.0 (1110.00 in binary 2's complement) becomes an output of 56 (111000 in binary)."
  reinterpret2 : xbsIndex_r4/Reinterpret  force_arith_type=on  arith_type=Unsigned  force_bin_pt=on  bin_pt=0  block_type=reinterpret
      settings: infoedit="Changes signal type without altering the binary representation.   You can changed the signal between signed and unsigned, and relocate the binary point.<br><br>Hardware notes: In hardware this block costs nothing.<br><br>Example:  Suppose the input is 6 bits wide, signed, with 2 fractional bits, and the output is forced to unsigned with 0 fractional bits.  Then an input of -2.0 (1110.00 in binary 2's complement) becomes an output of 56 (111000 in binary)."
  bus_out : Outport
  wires:
  reinterpret2/1 -> concatenate/2
  in2/1 -> reinterpret2/1
  reinterpret1/1 -> concatenate/1
  in1/1 -> reinterpret1/1
  concatenate/1 -> bus_out/1

== system r2_b8a4x1kf/sys0/bf/fbf/apply_beam_weights/munge_in/split ==
  bus_in : Inport
  reinterpret1 : xbsIndex_r4/Reinterpret  force_arith_type=on  arith_type=Unsigned  force_bin_pt=on  bin_pt=0  block_type=reinterpret
  reinterpret2 : xbsIndex_r4/Reinterpret  force_arith_type=on  arith_type=Unsigned  force_bin_pt=on  bin_pt=0  block_type=reinterpret
  slice1 : xbsIndex_r4/Slice  nbits=16  boolean_output=off  mode=Upper Bit Location + Width  bit1=-16  base1=MSB of Input  bit0=0  base0=LSB of Input  dbl_ovrd=off  block_type=slice
  slice2 : xbsIndex_r4/Slice  nbits=16  boolean_output=off  mode=Upper Bit Location + Width  bit1=0  base1=MSB of Input  bit0=0  base0=LSB of Input  dbl_ovrd=off  block_type=slice
  msb_out2 : Outport
  lsb_out1 : Outport  Port=2
  wires:
  bus_in/1 -> slice2/1, slice1/1
  slice2/1 -> reinterpret2/1
  reinterpret2/1 -> msb_out2/1
  slice1/1 -> reinterpret1/1
  reinterpret1/1 -> lsb_out1/1

== system r2_b8a4x1kf/sys0/bf/fbf/combine/acc/bus_add ==
  a : Inport
  b : Inport  Port=2
  misci : Inport  Port=3
  a_debus : Subsystem  AncestorBlock=casper_library_flow_control/bus_expand  mask(bus_expand){mode=divisions of arbitrary size, outputNum=1, outputWidth=[25  25  25  25], outputBinaryPt=[16  16  16  16], outputArithmeticType=[1  1  1  1], show_format=on, outputToWorkspace=off, variablePrefix=, outputToModelAsWell=on}
      mask prompts: outputNum "Number of outputs:"; outputWidth "Output width [msb ... lsb]:"; outputBinaryPt "Output binary point position [msb ... lsb]:"; outputArithmeticType "Output arithmetic type (ufix=0, fix=1, bool=2) [msb ... lsb]:"; show_format "Print format string?"; outputToWorkspace "Output to workspace?"; variablePrefix "Variable name prefix:"; outputToModelAsWell "Output to model as well?"
      mask help:
      | Expands a 'bus' made using a bus_create or Xilinx
      | concat block.
      | The input will be divided into the specified number
      | of outputs with the specified arithmetic types.
      | Divisions are made from most significant bit.
      mask init: same as r2_b8a4x1kf/bus_expand
      settings: AttributesFormatString=4 outputs: f25.16,f25.16,f25.16,f25.16,
      mask TypeOptions mode: divisions of equal size | divisions of arbitrary size
      mask Callback mode: bus_expand_callback();
      mask Callback outputWidth: bus_expand_callback();
      mask Callback outputToWorkspace: bus_expand_callback();
  addsub{1..4} (4 alike) : xbsIndex_r4/AddSub  mode=Addition  use_carryin=off  use_carryout=off  en=off  latency=3  precision=User Defined  arith_type="Signed  (2's comp)"  n_bits=28  bin_pt=16  quantization=Truncate  overflow=Wrap  dbl_ovrd=off  use_behavioral_HDL=off  hw_selection=Fabric  pipelined=on  block_type=addsub
  b_debus : Subsystem  AncestorBlock=casper_library_flow_control/bus_expand  mask(bus_expand){mode=divisions of arbitrary size, outputNum=1, outputWidth=[28  28  28  28], outputBinaryPt=[16  16  16  16], outputArithmeticType=[1  1  1  1], show_format=on, outputToWorkspace=off, variablePrefix=, outputToModelAsWell=on}
      mask prompts: outputNum "Number of outputs:"; outputWidth "Output width [msb ... lsb]:"; outputBinaryPt "Output binary point position [msb ... lsb]:"; outputArithmeticType "Output arithmetic type (ufix=0, fix=1, bool=2) [msb ... lsb]:"; show_format "Print format string?"; outputToWorkspace "Output to workspace?"; variablePrefix "Variable name prefix:"; outputToModelAsWell "Output to model as well?"
      mask help:
      | Expands a 'bus' made using a bus_create or Xilinx
      | concat block.
      | The input will be divided into the specified number
      | of outputs with the specified arithmetic types.
      | Divisions are made from most significant bit.
      mask init: same as r2_b8a4x1kf/bus_expand
      settings: AttributesFormatString=4 outputs: f28.16,f28.16,f28.16,f28.16,
      mask TypeOptions mode: divisions of equal size | divisions of arbitrary size
      mask Callback mode: bus_expand_callback();
      mask Callback outputWidth: bus_expand_callback();
      mask Callback outputToWorkspace: bus_expand_callback();
  dmisc : xbsIndex_r4/Delay  rst=off  infoeditControl=Selection of Reset will increase slice count due to use of real FFs and instead of SRLs  en=off  latency=3  dbl_ovrd=off  reg_retiming=off  block_type=delay
  op_bussify : Subsystem  AncestorBlock=casper_library_flow_control/bus_create  mask(bus_create){inputNum=4}
      mask prompts: inputNum "Number of inputs:"
      mask init:
      | bus_create_init(gcb,...
      |     'inputNum', inputNum);
  dout : Outport
  misco : Outport  Port=2
  wires:
  a/1 -> a_debus/1(bus_in)
  b/1 -> b_debus/1(bus_in)
  a_debus/1(msb_out4) -> addsub1/1
  b_debus/1(msb_out4) -> addsub1/2
  a_debus/2(out3) -> addsub2/1
  b_debus/2(out3) -> addsub2/2
  a_debus/3(out2) -> addsub3/1
  b_debus/3(out2) -> addsub3/2
  a_debus/4(lsb_out1) -> addsub4/1
  b_debus/4(lsb_out1) -> addsub4/2
  misci/1 -> dmisc/1
  addsub1/1 -> op_bussify/1(in1)
  addsub2/1 -> op_bussify/2(in2)
  addsub3/1 -> op_bussify/3(in3)
  addsub4/1 -> op_bussify/4(in4)
  op_bussify/1(bus_out) -> dout/1
  dmisc/1 -> misco/1

== system r2_b8a4x1kf/sys0/bf/fbf/combine/acc/bus_register ==
  din : Inport
  rst : Inport  Port=2
  misci : Inport  Port=3
  din_expand : Subsystem  AncestorBlock=casper_library_flow_control/bus_expand  mask(bus_expand){mode=divisions of arbitrary size, outputNum=1, outputWidth=[50  50], outputBinaryPt=[0  0], outputArithmeticType=[0  0], show_format=on, outputToWorkspace=off, variablePrefix=, outputToModelAsWell=on}
      mask prompts: outputNum "Number of outputs:"; outputWidth "Output width [msb ... lsb]:"; outputBinaryPt "Output binary point position [msb ... lsb]:"; outputArithmeticType "Output arithmetic type (ufix=0, fix=1, bool=2) [msb ... lsb]:"; show_format "Print format string?"; outputToWorkspace "Output to workspace?"; variablePrefix "Variable name prefix:"; outputToModelAsWell "Output to model as well?"
      mask help:
      | Expands a 'bus' made using a bus_create or Xilinx
      | concat block.
      | The input will be divided into the specified number
      | of outputs with the specified arithmetic types.
      | Divisions are made from most significant bit.
      mask init: same as r2_b8a4x1kf/bus_expand
      settings: AttributesFormatString=2 outputs: uf50.0,uf50.0,
      mask TypeOptions mode: divisions of equal size | divisions of arbitrary size
      mask Callback mode: bus_expand_callback();
      mask Callback outputWidth: bus_expand_callback();
      mask Callback outputToWorkspace: bus_expand_callback();
  dmisc : xbsIndex_r4/Delay  rst=off  infoeditControl=Selection of Reset will increase slice count due to use of real FFs and instead of SRLs  en=off  latency=1  dbl_ovrd=off  reg_retiming=on  block_type=delay
  dout_compress : Subsystem  AncestorBlock=casper_library_flow_control/bus_create  mask(bus_create){inputNum=2}
      mask prompts: inputNum "Number of inputs:"
      mask init:
      | bus_create_init(gcb,...
      |     'inputNum', inputNum);
  reg1 : xbsIndex_r4/Register  init=0  rst=on  en=off  dbl_ovrd=off  block_type=register
  reg2 : xbsIndex_r4/Register  init=0  rst=on  en=off  dbl_ovrd=off  block_type=register
  rst_expand : Subsystem  AncestorBlock=casper_library_flow_control/bus_expand  mask(bus_expand){mode=divisions of equal size, outputNum=2, outputWidth=1, outputBinaryPt=0, outputArithmeticType=2, show_format=on, outputToWorkspace=off, variablePrefix=, outputToModelAsWell=on}
      mask prompts: outputNum "Number of outputs:"; outputWidth "Output width:"; outputBinaryPt "Output binary point position:"; outputArithmeticType "Output arithmetic type (ufix=0, fix=1, bool=2):"; show_format "Print format string?"; outputToWorkspace "Output to workspace?"; variablePrefix "Variable name prefix:"; outputToModelAsWell "Output to model as well?"
      mask help:
      | Expands a 'bus' made using a bus_create or Xilinx
      | concat block.
      | The input will be divided into the specified number
      | of outputs with the specified arithmetic types.
      | Divisions are made from most significant bit.
      mask init: same as r2_b8a4x1kf/bus_expand
      settings: AttributesFormatString=2 outputs: b,b,
      mask TypeOptions mode: divisions of equal size | divisions of arbitrary size
      mask Callback mode: bus_expand_callback();
      mask Callback outputWidth: bus_expand_callback();
      mask Callback outputToWorkspace: bus_expand_callback();
  dout : Outport
  misco : Outport  Port=2
  wires:
  din/1 -> din_expand/1(bus_in)
  rst/1 -> rst_expand/1(bus_in)
  din_expand/1(msb_out2) -> reg1/1
  rst_expand/1(msb_out2) -> reg1/2
  din_expand/2(lsb_out1) -> reg2/1
  rst_expand/2(lsb_out1) -> reg2/2
  misci/1 -> dmisc/1
  reg1/1 -> dout_compress/1(in1)
  reg2/1 -> dout_compress/2(in2)
  dout_compress/1(bus_out) -> dout/1
  dmisc/1 -> misco/1

== system r2_b8a4x1kf/sys0/bf/fbf/combine/acc_ctrl/edge_detect ==
  in : Inport
  Delay : xbsIndex_r4/Delay  rst=off  infoeditControl=Selection of Reset will increase slice count due to use of real FFs and instead of SRLs  en=off  latency=1  dbl_ovrd=off  reg_retiming=off  block_type=delay
      settings: xl_area=[0, 0, 0, 0, 0, 0, 0]
  Inverter : xbsIndex_r4/Inverter  en=off  latency=0  dbl_ovrd=off  block_type=inv
      settings: xl_area=[0, 0, 0, 0, 0, 0, 0]
  edge_op : xbsIndex_r4/Logical  logical_function=NOR  inputs=2  en=off  latency=0  precision=Full  arith_type=Unsigned  n_bits=8  bin_pt=2  align_bp=on  dbl_ovrd=off  block_type=logical
      settings: xl_area=[0, 0, 0, 0, 0, 0, 0]
  out : Outport
  wires:
  Delay/1 -> edge_op/2
  in/1 -> Delay/1, Inverter/1
  edge_op/1 -> out/1
  Inverter/1 -> edge_op/1

== system r2_b8a4x1kf/sys0/bf/fbf/filter/en_replicate/bussify ==
  in1 : Inport
  in2 : Inport  Port=2
  concatenate : xbsIndex_r4/Concat  num_inputs=2  dbl_ovrd=off  block_type=concat
  reinterpret1 : xbsIndex_r4/Reinterpret  force_arith_type=on  arith_type=Unsigned  force_bin_pt=on  bin_pt=0  block_type=reinterpret
      settings: infoedit="Changes signal type without altering the binary representation.   You can changed the signal between signed and unsigned, and relocate the binary point.<br><br>Hardware notes: In hardware this block costs nothing.<br><br>Example:  Suppose the input is 6 bits wide, signed, with 2 fractional bits, and the output is forced to unsigned with 0 fractional bits.  Then an input of -2.0 (1110.00 in binary 2's complement) becomes an output of 56 (111000 in binary)."
  reinterpret2 : xbsIndex_r4/Reinterpret  force_arith_type=on  arith_type=Unsigned  force_bin_pt=on  bin_pt=0  block_type=reinterpret
      settings: infoedit="Changes signal type without altering the binary representation.   You can changed the signal between signed and unsigned, and relocate the binary point.<br><br>Hardware notes: In hardware this block costs nothing.<br><br>Example:  Suppose the input is 6 bits wide, signed, with 2 fractional bits, and the output is forced to unsigned with 0 fractional bits.  Then an input of -2.0 (1110.00 in binary 2's complement) becomes an output of 56 (111000 in binary)."
  bus_out : Outport
  wires:
  concatenate/1 -> bus_out/1
  in1/1 -> reinterpret1/1
  reinterpret1/1 -> concatenate/1
  in2/1 -> reinterpret2/1
  reinterpret2/1 -> concatenate/2

== system r2_b8a4x1kf/sys0/bf/fbf/filter/val_mux/d_bussify ==
  in1 : Inport
  reinterpret1 : xbsIndex_r4/Reinterpret  force_arith_type=on  arith_type=Unsigned  force_bin_pt=on  bin_pt=0  block_type=reinterpret
      settings: infoedit="Changes signal type without altering the binary representation.   You can changed the signal between signed and unsigned, and relocate the binary point.<br><br>Hardware notes: In hardware this block costs nothing.<br><br>Example:  Suppose the input is 6 bits wide, signed, with 2 fractional bits, and the output is forced to unsigned with 0 fractional bits.  Then an input of -2.0 (1110.00 in binary 2's complement) becomes an output of 56 (111000 in binary)."
  bus_out : Outport
  wires:
  reinterpret1/1 -> bus_out/1
  in1/1 -> reinterpret1/1
